simulink model "IEEE_BUS_68_AGC"  (R2025a)
settings: Solver=ode23tb  StartTime=0.0  StopTime=150  FixedStep=Ts  MaxStep=0.0001  RelTol=1e-3
PreLoadFcn:
  | PSSMODEL=1;
  | LPSS=0;
  | WAPSS=0;
  | WAPSS2=0;
  | Ts=50e-5;
InitFcn:
  | PSSMODEL=1;
  | LPSS=0;
  | WAPSS=0;
  | WAPSS2=0;
  | Ts=50e-5;
  | 
  | % Required data to 68 Bus benchmark
  | % clear
  | % clc
  | % Definition for the columns
  | % system base =100 MVA
  | 
  | %% Line data Format (line)
  | % All values are given on the same system base MVA
  | % 1: From bus
  | % 2: To bus
  | % 3: Resistance (pu)
  | % 4: Reactance  (pu)
  | % 5: Charge     (pu)
  | % 6: Transformer Tap Amplitute
  | % 7: base MVA
  | % 8: Nomonal Voltage (KV)
  | 
  | %1   2    3        4       5       6        7      8
  | line=[...
  | 1	54	0	     0.0181	  0	      1.025     100    13.8
  | 2	58	0	     0.025	  0	      1.070     100    13.8
  | 3	62	0	     0.02	  0	      1.070     100    13.8
  | 4	19	0.0007	 0.0142	  0	      1.070     100    13.8
  | 5	20	0.0009	 0.018	  0	      1.009     100    13.8
  | 6	22	0	     0.0143	  0	      1.025     100    13.8
  | 7	23	0.0005	 0.0272	  0	      0         100    13.8
  | 8	25	0.0006	 0.0232	  0	      1.025     100    13.8
  | 9	29	0.0008	 0.0156   0	      1.025     100    13.8
  | 10	31	0	     0.026	  0	      1.04      100    13.8
  | 11	32	0	     0.013	  0	      1.04      100    13.8
  | 12	36	0	     0.0075	  0	      1.04      100    13.8
  | 13	17	0	     0.0033	  0	      1.04      100    13.8
  | 14	41	0	     0.0015	  0	      1         100    13.8
  | 15	42	0	     0.0015	  0	      1         100    13.8
  | 16	18	0	     0.003	  0	      1         100    13.8
  | 17	36	0.0005	 0.0045	  0.32	  0         100    138
  | 17	43	0.0005	 0.0276	  0	      0         100    138
  | 18	42	0.004	 0.06	  2.25    0         100    138
  | 18	49	0.0076	 0.1141	  1.16    0	        100    138
  | 18	50	0.0012	 0.0288	  2.06	  0         100    138
  | 20	19	0.0007	 0.0138	  0       1.06	    100    138
  | 19	68	0.0016	 0.0195	  0.304	  0         100    138
  | 21	22	0.0008	 0.014	  0.2565  0	        100    138
  | 21	68	0.0008	 0.0135	  0.2548  0	        100    138
  | 22	23	0.0006	 0.0096	  0.1846  0	        100    138
  | 23	24	0.0022	 0.035	  0.361	  0         100    138
  | 24	68	0.0003	 0.0059	  0.068	  0         100    138
  | 25	26	0.0032	 0.0323	  0.531	  0         100    138
  | 25	54	0.007	 0.0086	  0.146	  0         100    138
  | 26	27	0.0014	 0.0147	  0.2396  0	        100    138
  | 26	28	0.0043	 0.0474	  0.7802  0	        100    138
  | 26	29	0.0057	 0.0625	  1.029	  0         100    138
  | 27	37	0.0013	 0.0173	  0.3216  0	        100    138
  | 27	53	0.032	 0.32	  0.41	  0         100    138
  | ... (+206 lines)
undefined symbols (not defined in the file or in its folder): D1, Delta
libraries: spsPMUPLLBasedPositiveSequenceLib x90, spsRMSLib x73, spsThreePhaseVIMeasurementLib x69, spsLoadFlowBusLib x69, spsThreePhasePISectionLineLib x64, spsThreePhaseParallelRLCLoadLib x35, spsGenericPowerSystemStabilizerLib x32, spsThreePhaseSeriesRLCLoadLib x21, spsThreePhaseTransformerTwoWindingsLib x21, spsSynchronousMachinepuStandardLib x20, spsExcitationSystemLib x16, spsMultiBandPowerSystemStabilizerLib x16
(part 8 of 8)

== system IEEE_BUS_68_AGC/area-4/G10/M10: Turbine & Regulators  ==
  note: M10
  m10 : Inport
  Pref10 : Inport  Port=2
  Vref10 : Inport  Port=3
  PSS10 : Inport  Port=4
  Bus Selector : BusSelector  OutputSignals="Mechanical.Rotor speed  wm  (pu),Mechanical.Rotor angle deviation  d_theta (rad),Mechanical.Electrical power  Pe (pu),Mechanical.Rotor speed deviation  dw (pu),Mechanical.Rotor mechanical angle  theta (deg),dq0 components.Stator voltage  vd (pu),dq0 components.Stator voltage  vq (pu),Output reactive power  Qeo (pu)"
  "Delta Pa PSS 10 " : spsGenericPowerSystemStabilizerLib/Generic Power System Stabilizer  Tsensor=15e-3  K=2.5*1.25  Twashout=1  Tleadlag1=[60e-3 1]  Tleadlag2=[0 0]  VSlimits=[-0.15 0.15]  Vinit=0  Plot_On=off  MagdB_On=on  FreqRange=logspace(-2,2,500)
      settings: LibrarySourceBlock=|
      | sps_lib/Electrical Machines/Synchronous Machine Control/Generic
      | Power System Stabilizer
  Delta w PSS (Kundur) 10 : spsGenericPowerSystemStabilizerLib/Generic Power System Stabilizer  Tsensor=15e-3  K=30  Twashout=10  Tleadlag1=[50e-3 20e-3]  Tleadlag2=[3 5.4]  VSlimits=[-0.15 0.15]  Vinit=0  Plot_On=off  MagdB_On=on  FreqRange=logspace(-2,2,500)
      settings: LibrarySourceBlock=|
      | sps_lib/Electrical Machines/Synchronous Machine Control/Generic
      | Power System Stabilizer
  EXCITATION10 : spsExcitationSystemLib/Excitation System  tr=AVR_Data(7,1)  reg=[ AVR_Data(7,2:3) ]  exc=[ 1, 0 ]  tgr=[ AVR_Data(7,4:5)]  damp=[ 0, 0 ]  sat=[ 0, 0 ]  lim="[ AVR_Data(7,7:8)  0 ]"  v0=[1.01 1.0142]
      settings: LibrarySourceBlock=sps_lib/Electrical Machines/Synchronous Machine Control/Excitation System
  MB-PSS10 : spsMultiBandPowerSystemStabilizerLib/Multi-Band Power System Stabilizer  OperationMode=Simplified settings  Kg=MB(1)  GL=[MB(2) MB(3)]  GI=[MB(4) MB(5)]  GH=[MB(6) MB(7)]  GLd=[66 66 9.4]  TcLF=[1.667 2 0 0 0 0 2 2.4 0 0 0 0 1 1]  GId=[66 66 47.6]  TcIF=[1 1 0.25 0.3 0 0 1 1 0.3 0.36 0 0 0 0]  GHd=[66 66 233]  TcHF="[0.01 0.012 0 0 0 0  0.012 0.0144 0 0 0 0 1 1]"  LIM=[.075 .15 .15 .15]  Plot_On=off  MagdB_On=off  FreqRange=logspace(-2,2,500)
      settings: LibrarySourceBlock=|
      | sps_lib/Electrical Machines/Synchronous Machine Control/Multi-Band
      | Power System Stabilizer
  Multiport Switch1 : MultiPortSwitch  Inputs=4  SaturateOnIntegerOverflow=off
  PSS model3 : Constant  Value=0
  PSS model4 : Constant
  Real-Imag to Complex1 : RealImagToComplex
  STG10 : spsSteamTurbineandGovernorLib/Steam Turbine and Governor  gentype=Tandem-compound (single mass)  reg1="[ 1  0.05    0 ]"  reg2="[ 0.001  0.15 ]"  reg3="[ -0.1  0.1  0  4.496 ]"  N=Ns  turb1="[ 0  10   3.3   0.5   ]"  turb2="[   0   0.36    0.36   0.28   ]"  HA="[ 0.046  1.430  1.465   0.192 ]"  KA="[ 90.44  53.88  64.59   62.94  ]"  DA="[ 0.0115  0.3575  0.3663   0.0137  ]"  ini1=0.5  ini2=[0.779316,-31.4247]
      settings: LibrarySourceBlock=|
      | sps_lib/Electrical Machines/Synchronous Machine Control/Steam Turbine
      | and Governor
  Sum2 : Sum  InputSameDT=on  SaturateOnIntegerOverflow=on  OutDataTypeStr=Inherit: Same as first input
  Sum3 : Sum  Inputs=-+  InputSameDT=on  SaturateOnIntegerOverflow=on  OutDataTypeStr=Inherit: Same as first input
  Terminator3 : Terminator
  Terminator4 : Terminator
  Terminator5 : Terminator
  wref10 : Constant
  Pm10 : Outport  InitialOutput=0
  Vf10 : Outport  Port=2  InitialOutput=0
  tag scope: EFD10=global, Pa10=global, Pe10=global, Q10=global, Vt10=global, d_theta10=global, pss10=global, theta10=global, w10=global
  wires:
  PSS10/1 -> Sum2/1
  Multiport Switch1/1 -> EXCITATION10/4, [pss10]
  PSS model3/1 -> Multiport Switch1/2
  MB-PSS10/1 -> Multiport Switch1/3
  Delta w PSS (Kundur) 10/1 -> Multiport Switch1/4
  "Delta Pa PSS 10 "/1 -> Multiport Switch1/5
  PSS model4/1 -> Sum2/2
  Sum2/1 -> Multiport Switch1/1
  Sum3/1 -> "Delta Pa PSS 10 "/1, [Pa10]  "Pm-Pe"
  Bus Selector/8 -> [Q10]  "<Output reactive power  Qeo (pu)>"
  Bus Selector/4 -> MB-PSS10/1, Delta w PSS (Kundur) 10/1  "<Rotor speed deviation  dw (pu)>"
  Bus Selector/3 -> [Pe10], Sum3/1  "<Electrical power  Pe (pu)>"
  Bus Selector/2 -> [d_theta10], STG10/4  "<Rotor angle deviation  d_theta (rad)>"
  Bus Selector/1 -> STG10/3, [w10]  "<Rotor speed  wm  (pu)>"
  STG10/1 -> Terminator5/1
  STG10/2 -> Terminator4/1
  STG10/4 -> Pm10/1, Sum3/2
  STG10/3 -> Terminator3/1
  Bus Selector/6 -> Real-Imag to Complex1/1, EXCITATION10/2  "<Stator voltage  vd (pu)>"
  Bus Selector/5 -> [theta10]  "<Rotor mechanical angle  theta (deg)>"
  Real-Imag to Complex1/1 -> [Vt10]
  EXCITATION10/1 -> [EFD10], Vf10/1
  Vref10/1 -> EXCITATION10/1
  m10/1 -> Bus Selector/1
  Pref10/1 -> STG10/2
  wref10/1 -> STG10/1
  Bus Selector/7 -> Real-Imag to Complex1/2, EXCITATION10/3  "<Stator voltage  vq (pu)>"

== system IEEE_BUS_68_AGC/area-4/G11/M11: Turbine & Regulators  ==
  note: M11
  m11 : Inport
  Pref11 : Inport  Port=2
  Vref11 : Inport  Port=3
  PSS11 : Inport  Port=4
  Bus Selector : BusSelector  OutputSignals="Mechanical.Rotor speed  wm  (pu),Mechanical.Rotor angle deviation  d_theta (rad),Mechanical.Electrical power  Pe (pu),Mechanical.Rotor speed deviation  dw (pu),Mechanical.Rotor mechanical angle  theta (deg),dq0 components.Stator voltage  vd (pu),dq0 components.Stator voltage  vq (pu),Output reactive power  Qeo (pu)"
  "Delta Pa PSS 11 " : spsGenericPowerSystemStabilizerLib/Generic Power System Stabilizer  Tsensor=15e-3  K=2.5*1.25  Twashout=1  Tleadlag1=[60e-3 1]  Tleadlag2=[0 0]  VSlimits=[-0.15 0.15]  Vinit=0  Plot_On=off  MagdB_On=on  FreqRange=logspace(-2,2,500)
      settings: LibrarySourceBlock=|
      | sps_lib/Electrical Machines/Synchronous Machine Control/Generic
      | Power System Stabilizer
  Delta w PSS (Kundur) 11 : spsGenericPowerSystemStabilizerLib/Generic Power System Stabilizer  Tsensor=15e-3  K=30  Twashout=10  Tleadlag1=[50e-3 20e-3]  Tleadlag2=[3 5.4]  VSlimits=[-0.15 0.15]  Vinit=0  Plot_On=off  MagdB_On=on  FreqRange=logspace(-2,2,500)
      settings: LibrarySourceBlock=|
      | sps_lib/Electrical Machines/Synchronous Machine Control/Generic
      | Power System Stabilizer
  EXCITATION11 : spsExcitationSystemLib/Excitation System  tr=AVR_Data(11,1)  reg=[ AVR_Data(11,2:3) ]  exc=[ 1, 0 ]  tgr=[ AVR_Data(11,4:5)]  damp=[ 0, 0 ]  sat=[ 0, 0 ]  lim="[ AVR_Data(11,7:8)  0 ]"  v0=[1 1.0051]
      settings: LibrarySourceBlock=sps_lib/Electrical Machines/Synchronous Machine Control/Excitation System
  MB-PSS11 : spsMultiBandPowerSystemStabilizerLib/Multi-Band Power System Stabilizer  OperationMode=Simplified settings  Kg=MB(1)  GL=[MB(2) MB(3)]  GI=[MB(4) MB(5)]  GH=[MB(6) MB(7)]  GLd=[66 66 9.4]  TcLF=[1.667 2 0 0 0 0 2 2.4 0 0 0 0 1 1]  GId=[66 66 47.6]  TcIF=[1 1 0.25 0.3 0 0 1 1 0.3 0.36 0 0 0 0]  GHd=[66 66 233]  TcHF="[0.01 0.012 0 0 0 0  0.012 0.0144 0 0 0 0 1 1]"  LIM=[.075 .15 .15 .15]  Plot_On=off  MagdB_On=off  FreqRange=logspace(-2,2,500)
      settings: LibrarySourceBlock=|
      | sps_lib/Electrical Machines/Synchronous Machine Control/Multi-Band
      | Power System Stabilizer
  Multiport Switch1 : MultiPortSwitch  Inputs=4  SaturateOnIntegerOverflow=off
  PSS model3 : Constant  Value=0
  PSS model4 : Constant
  Real-Imag to Complex1 : RealImagToComplex
  STG11 : spsSteamTurbineandGovernorLib/Steam Turbine and Governor  gentype=Tandem-compound (single mass)  reg1="[ 1  0.05    0 ]"  reg2="[ 0.001  0.15 ]"  reg3="[ -0.1  0.1  0  4.496 ]"  N=Ns  turb1="[ 0  10   3.3   0.5   ]"  turb2="[   0   0.36    0.36   0.28   ]"  HA="[ 0.046  1.430  1.465   0.192 ]"  KA="[ 90.44  53.88  64.59   62.94  ]"  DA="[ 0.0115  0.3575  0.3663   0.0137  ]"  ini1=0.5  ini2=[0.779316,-31.4247]
      settings: LibrarySourceBlock=|
      | sps_lib/Electrical Machines/Synchronous Machine Control/Steam Turbine
      | and Governor
  Sum2 : Sum  InputSameDT=on  SaturateOnIntegerOverflow=on  OutDataTypeStr=Inherit: Same as first input
  Sum3 : Sum  Inputs=-+  InputSameDT=on  SaturateOnIntegerOverflow=on  OutDataTypeStr=Inherit: Same as first input
  Terminator3 : Terminator
  Terminator4 : Terminator
  Terminator5 : Terminator
  wref11 : Constant
  Pm11 : Outport  InitialOutput=0
  Vf11 : Outport  Port=2  InitialOutput=0
  tag scope: EFD11=global, Pa11=global, Pe11=global, Q11=global, Vt11=global, d_theta11=global, pss11=global, theta11=global, w11=global
  wires:
  Bus Selector/7 -> EXCITATION11/3, Real-Imag to Complex1/2  "<Stator voltage  vq (pu)>"
  wref11/1 -> STG11/1
  Pref11/1 -> STG11/2
  m11/1 -> Bus Selector/1
  Vref11/1 -> EXCITATION11/1
  EXCITATION11/1 -> Vf11/1, [EFD11]
  Real-Imag to Complex1/1 -> [Vt11]
  Bus Selector/5 -> [theta11]  "<Rotor mechanical angle  theta (deg)>"
  Bus Selector/6 -> EXCITATION11/2, Real-Imag to Complex1/1  "<Stator voltage  vd (pu)>"
  STG11/3 -> Terminator3/1
  STG11/4 -> Sum3/2, Pm11/1
  STG11/2 -> Terminator4/1
  STG11/1 -> Terminator5/1
  Bus Selector/1 -> [w11], STG11/3  "<Rotor speed  wm  (pu)>"
  Bus Selector/2 -> STG11/4, [d_theta11]  "<Rotor angle deviation  d_theta (rad)>"
  Bus Selector/3 -> Sum3/1, [Pe11]  "<Electrical power  Pe (pu)>"
  Bus Selector/4 -> Delta w PSS (Kundur) 11/1, MB-PSS11/1  "<Rotor speed deviation  dw (pu)>"
  Bus Selector/8 -> [Q11]  "<Output reactive power  Qeo (pu)>"
  Sum3/1 -> [Pa11], "Delta Pa PSS 11 "/1  "Pm-Pe"
  Sum2/1 -> Multiport Switch1/1
  PSS model4/1 -> Sum2/2
  "Delta Pa PSS 11 "/1 -> Multiport Switch1/5
  Delta w PSS (Kundur) 11/1 -> Multiport Switch1/4
  MB-PSS11/1 -> Multiport Switch1/3
  PSS model3/1 -> Multiport Switch1/2
  Multiport Switch1/1 -> [pss11], EXCITATION11/4
  PSS11/1 -> Sum2/1

== system IEEE_BUS_68_AGC/area-4/G12/M12: Turbine & Regulators  ==
  note: M12
  m12 : Inport
  Pref12 : Inport  Port=2
  Vref12 : Inport  Port=3
  PSS12 : Inport  Port=4
  Bus Selector : BusSelector  OutputSignals="Mechanical.Rotor speed  wm  (pu),Mechanical.Rotor angle deviation  d_theta (rad),Mechanical.Electrical power  Pe (pu),Mechanical.Rotor speed deviation  dw (pu),Mechanical.Rotor mechanical angle  theta (deg),dq0 components.Stator voltage  vd (pu),dq0 components.Stator voltage  vq (pu),Output reactive power  Qeo (pu)"
  "Delta Pa PSS 12 " : spsGenericPowerSystemStabilizerLib/Generic Power System Stabilizer  Tsensor=15e-3  K=2.5*1.25  Twashout=1  Tleadlag1=[60e-3 1]  Tleadlag2=[0 0]  VSlimits=[-0.15 0.15]  Vinit=0  Plot_On=off  MagdB_On=on  FreqRange=logspace(-2,2,500)
      settings: LibrarySourceBlock=|
      | sps_lib/Electrical Machines/Synchronous Machine Control/Generic
      | Power System Stabilizer
  Delta w PSS (Kundur) 12 : spsGenericPowerSystemStabilizerLib/Generic Power System Stabilizer  Tsensor=15e-3  K=30  Twashout=10  Tleadlag1=[50e-3 20e-3]  Tleadlag2=[3 5.4]  VSlimits=[-0.15 0.15]  Vinit=0  Plot_On=off  MagdB_On=on  FreqRange=logspace(-2,2,500)
      settings: LibrarySourceBlock=|
      | sps_lib/Electrical Machines/Synchronous Machine Control/Generic
      | Power System Stabilizer
  EXCITATION12 : spsExcitationSystemLib/Excitation System  tr=AVR_Data(13,1)  reg=[ AVR_Data(13,2:3) ]  exc=[ 1, 0 ]  tgr=[ AVR_Data(13,4:5)]  damp=[ 0, 0 ]  sat=[ 0, 0 ]  lim="[ AVR_Data(13,7:8)  0 ]"  v0=[1.0156 1.0136]
      settings: LibrarySourceBlock=sps_lib/Electrical Machines/Synchronous Machine Control/Excitation System
  MB-PSS12 : spsMultiBandPowerSystemStabilizerLib/Multi-Band Power System Stabilizer  OperationMode=Simplified settings  Kg=MB(1)  GL=[MB(2) MB(3)]  GI=[MB(4) MB(5)]  GH=[MB(6) MB(7)]  GLd=[66 66 9.4]  TcLF=[1.667 2 0 0 0 0 2 2.4 0 0 0 0 1 1]  GId=[66 66 47.6]  TcIF=[1 1 0.25 0.3 0 0 1 1 0.3 0.36 0 0 0 0]  GHd=[66 66 233]  TcHF="[0.01 0.012 0 0 0 0  0.012 0.0144 0 0 0 0 1 1]"  LIM=[.075 .15 .15 .15]  Plot_On=off  MagdB_On=off  FreqRange=logspace(-2,2,500)
      settings: LibrarySourceBlock=|
      | sps_lib/Electrical Machines/Synchronous Machine Control/Multi-Band
      | Power System Stabilizer
  Multiport Switch1 : MultiPortSwitch  Inputs=4  SaturateOnIntegerOverflow=off
  PSS model3 : Constant  Value=0
  PSS model4 : Constant
  Real-Imag to Complex1 : RealImagToComplex
  STG12 : spsSteamTurbineandGovernorLib/Steam Turbine and Governor  gentype=Tandem-compound (single mass)  reg1="[ 1  0.05    0 ]"  reg2="[ 0.001  0.15 ]"  reg3="[ -0.1  0.1  0  4.496 ]"  N=Ns  turb1="[ 0  10   3.3   0.5   ]"  turb2="[   0   0.36    0.36   0.28   ]"  HA="[ 0.046  1.430  1.465   0.192 ]"  KA="[ 90.44  53.88  64.59   62.94  ]"  DA="[ 0.0115  0.3575  0.3663   0.0137  ]"  ini1=0.45  ini2=[0.779316,-31.4247]
      settings: LibrarySourceBlock=|
      | sps_lib/Electrical Machines/Synchronous Machine Control/Steam Turbine
      | and Governor
  Sum2 : Sum  InputSameDT=on  SaturateOnIntegerOverflow=on  OutDataTypeStr=Inherit: Same as first input
  Sum3 : Sum  Inputs=-+  InputSameDT=on  SaturateOnIntegerOverflow=on  OutDataTypeStr=Inherit: Same as first input
  Terminator3 : Terminator
  Terminator4 : Terminator
  Terminator5 : Terminator
  wref12 : Constant
  Pm12 : Outport  InitialOutput=0
  Vf12 : Outport  Port=2  InitialOutput=0
  tag scope: EFD12=global, Pa12=global, Pe12=global, Q12=global, Vt12=global, d_theta12=global, pss12=global, theta12=global, w12=global
  wires:
  PSS12/1 -> Sum2/1
  Multiport Switch1/1 -> EXCITATION12/4, [pss12]
  PSS model3/1 -> Multiport Switch1/2
  MB-PSS12/1 -> Multiport Switch1/3
  Delta w PSS (Kundur) 12/1 -> Multiport Switch1/4
  "Delta Pa PSS 12 "/1 -> Multiport Switch1/5
  PSS model4/1 -> Sum2/2
  Sum2/1 -> Multiport Switch1/1
  Sum3/1 -> "Delta Pa PSS 12 "/1, [Pa12]  "Pm-Pe"
  Bus Selector/8 -> [Q12]  "<Output reactive power  Qeo (pu)>"
  Bus Selector/4 -> MB-PSS12/1, Delta w PSS (Kundur) 12/1  "<Rotor speed deviation  dw (pu)>"
  Bus Selector/3 -> [Pe12], Sum3/1  "<Electrical power  Pe (pu)>"
  Bus Selector/2 -> [d_theta12], STG12/4  "<Rotor angle deviation  d_theta (rad)>"
  Bus Selector/1 -> STG12/3, [w12]  "<Rotor speed  wm  (pu)>"
  STG12/1 -> Terminator5/1
  STG12/2 -> Terminator4/1
  STG12/4 -> Pm12/1, Sum3/2
  STG12/3 -> Terminator3/1
  Bus Selector/6 -> Real-Imag to Complex1/1, EXCITATION12/2  "<Stator voltage  vd (pu)>"
  Bus Selector/5 -> [theta12]  "<Rotor mechanical angle  theta (deg)>"
  Real-Imag to Complex1/1 -> [Vt12]
  EXCITATION12/1 -> [EFD12], Vf12/1
  Vref12/1 -> EXCITATION12/1
  m12/1 -> Bus Selector/1
  Pref12/1 -> STG12/2
  wref12/1 -> STG12/1
  Bus Selector/7 -> Real-Imag to Complex1/2, EXCITATION12/3  "<Stator voltage  vq (pu)>"

== system IEEE_BUS_68_AGC/area-4/G13/M13: Turbine & Regulators  ==
  note: M13
  m13 : Inport
  Pref13 : Inport  Port=2
  Vref13 : Inport  Port=3
  PSS13 : Inport  Port=4
  Bus Selector : BusSelector  OutputSignals="Mechanical.Rotor speed  wm  (pu),Mechanical.Rotor angle deviation  d_theta (rad),Mechanical.Electrical power  Pe (pu),Mechanical.Rotor speed deviation  dw (pu),Mechanical.Rotor mechanical angle  theta (deg),dq0 components.Stator voltage  vd (pu),dq0 components.Stator voltage  vq (pu),Output reactive power  Qeo (pu)"
  "Delta Pa PSS 13 " : spsGenericPowerSystemStabilizerLib/Generic Power System Stabilizer  Tsensor=15e-3  K=2.5*1.25  Twashout=1  Tleadlag1=[60e-3 1]  Tleadlag2=[0 0]  VSlimits=[-0.15 0.15]  Vinit=0  Plot_On=off  MagdB_On=on  FreqRange=logspace(-2,2,500)
      settings: LibrarySourceBlock=|
      | sps_lib/Electrical Machines/Synchronous Machine Control/Generic
      | Power System Stabilizer
  Delta w PSS (Kundur) 13 : spsGenericPowerSystemStabilizerLib/Generic Power System Stabilizer  Tsensor=15e-3  K=30  Twashout=10  Tleadlag1=[50e-3 20e-3]  Tleadlag2=[3 5.4]  VSlimits=[-0.15 0.15]  Vinit=0  Plot_On=off  MagdB_On=on  FreqRange=logspace(-2,2,500)
      settings: LibrarySourceBlock=|
      | sps_lib/Electrical Machines/Synchronous Machine Control/Generic
      | Power System Stabilizer
  EXCITATION13 : spsExcitationSystemLib/Excitation System  tr=AVR_Data(13,1)  reg=[ AVR_Data(13,2:3) ]  exc=[ 1, 0 ]  tgr=[ AVR_Data(13,4:5)]  damp=[ 0, 0 ]  sat=[ 0, 0 ]  lim="[ AVR_Data(13,7:8)  0 ]"  v0=[1.011 1.016]
      settings: LibrarySourceBlock=sps_lib/Electrical Machines/Synchronous Machine Control/Excitation System
  MB-PSS13 : spsMultiBandPowerSystemStabilizerLib/Multi-Band Power System Stabilizer  OperationMode=Simplified settings  Kg=MB(1)  GL=[MB(2) MB(3)]  GI=[MB(4) MB(5)]  GH=[MB(6) MB(7)]  GLd=[66 66 9.4]  TcLF=[1.667 2 0 0 0 0 2 2.4 0 0 0 0 1 1]  GId=[66 66 47.6]  TcIF=[1 1 0.25 0.3 0 0 1 1 0.3 0.36 0 0 0 0]  GHd=[66 66 233]  TcHF="[0.01 0.012 0 0 0 0  0.012 0.0144 0 0 0 0 1 1]"  LIM=[.075 .15 .15 .15]  Plot_On=off  MagdB_On=off  FreqRange=logspace(-2,2,500)
      settings: LibrarySourceBlock=|
      | sps_lib/Electrical Machines/Synchronous Machine Control/Multi-Band
      | Power System Stabilizer
  Multiport Switch1 : MultiPortSwitch  Inputs=4  SaturateOnIntegerOverflow=off
  PSS model3 : Constant  Value=0
  PSS model4 : Constant
  Real-Imag to Complex1 : RealImagToComplex
  STG13 : spsSteamTurbineandGovernorLib/Steam Turbine and Governor  gentype=Tandem-compound (single mass)  reg1="[ 1  0.05    0 ]"  reg2="[ 0.001  0.15 ]"  reg3="[ -0.1  0.1  0  4.496 ]"  N=Ns  turb1="[ 0  10   3.3   0.5   ]"  turb2="[   0   0.36    0.36   0.28   ]"  HA="[ 0.046  1.430  1.465   0.192 ]"  KA="[ 90.44  53.88  64.59   62.94  ]"  DA="[ 0.0115  0.3575  0.3663   0.0137  ]"  ini1=0.5985  ini2=[0.779316,-31.4247]
      settings: LibrarySourceBlock=|
      | sps_lib/Electrical Machines/Synchronous Machine Control/Steam Turbine
      | and Governor
  Sum2 : Sum  InputSameDT=on  SaturateOnIntegerOverflow=on  OutDataTypeStr=Inherit: Same as first input
  Sum3 : Sum  Inputs=-+  InputSameDT=on  SaturateOnIntegerOverflow=on  OutDataTypeStr=Inherit: Same as first input
  Terminator3 : Terminator
  Terminator4 : Terminator
  Terminator5 : Terminator
  wref13 : Constant
  Pm13 : Outport  InitialOutput=0
  Vf13 : Outport  Port=2  InitialOutput=0
  tag scope: EFD13=global, Pa13=global, Pe13=global, Q13=global, Vt13=global, d_theta13=global, pss13=global, theta13=global, w13=global
  wires:
  Bus Selector/7 -> EXCITATION13/3, Real-Imag to Complex1/2  "<Stator voltage  vq (pu)>"
  wref13/1 -> STG13/1
  Pref13/1 -> STG13/2
  m13/1 -> Bus Selector/1
  Vref13/1 -> EXCITATION13/1
  EXCITATION13/1 -> Vf13/1, [EFD13]
  Real-Imag to Complex1/1 -> [Vt13]
  Bus Selector/5 -> [theta13]  "<Rotor mechanical angle  theta (deg)>"
  Bus Selector/6 -> EXCITATION13/2, Real-Imag to Complex1/1  "<Stator voltage  vd (pu)>"
  STG13/3 -> Terminator3/1
  STG13/4 -> Sum3/2, Pm13/1
  STG13/2 -> Terminator4/1
  STG13/1 -> Terminator5/1
  Bus Selector/1 -> [w13], STG13/3  "<Rotor speed  wm  (pu)>"
  Bus Selector/2 -> STG13/4, [d_theta13]  "<Rotor angle deviation  d_theta (rad)>"
  Bus Selector/3 -> Sum3/1, [Pe13]  "<Electrical power  Pe (pu)>"
  Bus Selector/4 -> Delta w PSS (Kundur) 13/1, MB-PSS13/1  "<Rotor speed deviation  dw (pu)>"
  Bus Selector/8 -> [Q13]  "<Output reactive power  Qeo (pu)>"
  Sum3/1 -> [Pa13], "Delta Pa PSS 13 "/1  "Pm-Pe"
  Sum2/1 -> Multiport Switch1/1
  PSS model4/1 -> Sum2/2
  "Delta Pa PSS 13 "/1 -> Multiport Switch1/5
  Delta w PSS (Kundur) 13/1 -> Multiport Switch1/4
  MB-PSS13/1 -> Multiport Switch1/3
  PSS model3/1 -> Multiport Switch1/2
  Multiport Switch1/1 -> [pss13], EXCITATION13/4
  PSS13/1 -> Sum2/1

== system IEEE_BUS_68_AGC/area-5/G14/M14: Turbine & Regulators  ==
  note: M14
  m14 : Inport
  Pref14 : Inport  Port=2
  Vref14 : Inport  Port=3
  PSS14 : Inport  Port=4
  Bus Selector : BusSelector  OutputSignals="Mechanical.Rotor speed  wm  (pu),Mechanical.Rotor angle deviation  d_theta (rad),Mechanical.Electrical power  Pe (pu),Mechanical.Rotor speed deviation  dw (pu),Mechanical.Rotor mechanical angle  theta (deg),dq0 components.Stator voltage  vd (pu),dq0 components.Stator voltage  vq (pu),Output reactive power  Qeo (pu)"
  "Delta Pa PSS 14 " : spsGenericPowerSystemStabilizerLib/Generic Power System Stabilizer  Tsensor=15e-3  K=2.5*1.25  Twashout=1  Tleadlag1=[60e-3 1]  Tleadlag2=[0 0]  VSlimits=[-0.15 0.15]  Vinit=0  Plot_On=off  MagdB_On=on  FreqRange=logspace(-2,2,500)
      settings: LibrarySourceBlock=|
      | sps_lib/Electrical Machines/Synchronous Machine Control/Generic
      | Power System Stabilizer
  Delta w PSS (Kundur) 14 : spsGenericPowerSystemStabilizerLib/Generic Power System Stabilizer  Tsensor=15e-3  K=30  Twashout=10  Tleadlag1=[50e-3 20e-3]  Tleadlag2=[3 5.4]  VSlimits=[-0.15 0.15]  Vinit=0  Plot_On=off  MagdB_On=on  FreqRange=logspace(-2,2,500)
      settings: LibrarySourceBlock=|
      | sps_lib/Electrical Machines/Synchronous Machine Control/Generic
      | Power System Stabilizer
  EXCITATION14 : spsExcitationSystemLib/Excitation System  tr=AVR_Data(14,1)  reg=[ AVR_Data(14,2:3) ]  exc=[ 1, 0 ]  tgr=[ AVR_Data(14,4:5)]  damp=[ 0, 0 ]  sat=[ 0, 0 ]  lim="[ AVR_Data(14,7:8)  0 ]"  v0=[1 1.0004]
      settings: LibrarySourceBlock=sps_lib/Electrical Machines/Synchronous Machine Control/Excitation System
  MB-PSS14 : spsMultiBandPowerSystemStabilizerLib/Multi-Band Power System Stabilizer  OperationMode=Simplified settings  Kg=MB(1)  GL=[MB(2) MB(3)]  GI=[MB(4) MB(5)]  GH=[MB(6) MB(7)]  GLd=[66 66 9.4]  TcLF=[1.667 2 0 0 0 0 2 2.4 0 0 0 0 1 1]  GId=[66 66 47.6]  TcIF=[1 1 0.25 0.3 0 0 1 1 0.3 0.36 0 0 0 0]  GHd=[66 66 233]  TcHF="[0.01 0.012 0 0 0 0  0.012 0.0144 0 0 0 0 1 1]"  LIM=[.075 .15 .15 .15]  Plot_On=off  MagdB_On=off  FreqRange=logspace(-2,2,500)
      settings: LibrarySourceBlock=|
      | sps_lib/Electrical Machines/Synchronous Machine Control/Multi-Band
      | Power System Stabilizer
  Multiport Switch1 : MultiPortSwitch  Inputs=4  SaturateOnIntegerOverflow=off
  PSS model3 : Constant  Value=0
  PSS model4 : Constant
  Real-Imag to Complex1 : RealImagToComplex
  STG14 : spsSteamTurbineandGovernorLib/Steam Turbine and Governor  gentype=Tandem-compound (single mass)  reg1="[ 1  0.05    0 ]"  reg2="[ 0.001  0.15 ]"  reg3="[ -0.1  0.1  0  4.496 ]"  N=Ns  turb1="[ 0  10   3.3   0.5   ]"  turb2="[   0   0.36    0.36   0.28   ]"  HA="[ 0.046  1.430  1.465   0.192 ]"  KA="[ 90.44  53.88  64.59   62.94  ]"  DA="[ 0.0115  0.3575  0.3663   0.0137  ]"  ini1=0.595  ini2=[0.779316,-31.4247]
      settings: LibrarySourceBlock=|
      | sps_lib/Electrical Machines/Synchronous Machine Control/Steam Turbine
      | and Governor
  Sum2 : Sum  InputSameDT=on  SaturateOnIntegerOverflow=on  OutDataTypeStr=Inherit: Same as first input
  Sum3 : Sum  Inputs=-+  InputSameDT=on  SaturateOnIntegerOverflow=on  OutDataTypeStr=Inherit: Same as first input
  Terminator3 : Terminator
  Terminator4 : Terminator
  Terminator5 : Terminator
  wref14 : Constant
  Pm14 : Outport  InitialOutput=0
  Vf14 : Outport  Port=2  InitialOutput=0
  tag scope: EFD14=global, Pa14=global, Pe14=global, Q14=global, Vt14=global, d_theta14=global, pss14=global, theta14=global, w14=global
  wires:
  PSS14/1 -> Sum2/1
  Multiport Switch1/1 -> EXCITATION14/4, [pss14]
  PSS model3/1 -> Multiport Switch1/2
  MB-PSS14/1 -> Multiport Switch1/3
  Delta w PSS (Kundur) 14/1 -> Multiport Switch1/4
  "Delta Pa PSS 14 "/1 -> Multiport Switch1/5
  PSS model4/1 -> Sum2/2
  Sum2/1 -> Multiport Switch1/1
  Sum3/1 -> "Delta Pa PSS 14 "/1, [Pa14]  "Pm-Pe"
  Bus Selector/8 -> [Q14]  "<Output reactive power  Qeo (pu)>"
  Bus Selector/4 -> MB-PSS14/1, Delta w PSS (Kundur) 14/1  "<Rotor speed deviation  dw (pu)>"
  Bus Selector/3 -> [Pe14], Sum3/1  "<Electrical power  Pe (pu)>"
  Bus Selector/2 -> [d_theta14], STG14/4  "<Rotor angle deviation  d_theta (rad)>"
  Bus Selector/1 -> STG14/3, [w14]  "<Rotor speed  wm  (pu)>"
  STG14/1 -> Terminator5/1
  STG14/2 -> Terminator4/1
  STG14/4 -> Pm14/1, Sum3/2
  STG14/3 -> Terminator3/1
  Bus Selector/6 -> Real-Imag to Complex1/1, EXCITATION14/2  "<Stator voltage  vd (pu)>"
  Bus Selector/5 -> [theta14]  "<Rotor mechanical angle  theta (deg)>"
  Real-Imag to Complex1/1 -> [Vt14]
  EXCITATION14/1 -> [EFD14], Vf14/1
  Vref14/1 -> EXCITATION14/1
  m14/1 -> Bus Selector/1
  Pref14/1 -> STG14/2
  wref14/1 -> STG14/1
  Bus Selector/7 -> Real-Imag to Complex1/2, EXCITATION14/3  "<Stator voltage  vq (pu)>"

== system IEEE_BUS_68_AGC/area-5/G15/M15: Turbine & Regulators  ==
  note: M15
  m15 : Inport
  Pref15 : Inport  Port=2
  Vref15 : Inport  Port=3
  PSS15 : Inport  Port=4
  Bus Selector : BusSelector  OutputSignals="Mechanical.Rotor speed  wm  (pu),Mechanical.Rotor angle deviation  d_theta (rad),Mechanical.Electrical power  Pe (pu),Mechanical.Rotor speed deviation  dw (pu),Mechanical.Rotor mechanical angle  theta (deg),dq0 components.Stator voltage  vd (pu),dq0 components.Stator voltage  vq (pu),Output reactive power  Qeo (pu)"
  "Delta Pa PSS 15 " : spsGenericPowerSystemStabilizerLib/Generic Power System Stabilizer  Tsensor=15e-3  K=2.5*1.25  Twashout=1  Tleadlag1=[60e-3 1]  Tleadlag2=[0 0]  VSlimits=[-0.15 0.15]  Vinit=0  Plot_On=off  MagdB_On=on  FreqRange=logspace(-2,2,500)
      settings: LibrarySourceBlock=|
      | sps_lib/Electrical Machines/Synchronous Machine Control/Generic
      | Power System Stabilizer
  Delta w PSS (Kundur) 15 : spsGenericPowerSystemStabilizerLib/Generic Power System Stabilizer  Tsensor=15e-3  K=30  Twashout=10  Tleadlag1=[50e-3 20e-3]  Tleadlag2=[3 5.4]  VSlimits=[-0.15 0.15]  Vinit=0  Plot_On=off  MagdB_On=on  FreqRange=logspace(-2,2,500)
      settings: LibrarySourceBlock=|
      | sps_lib/Electrical Machines/Synchronous Machine Control/Generic
      | Power System Stabilizer
  EXCITATION15 : spsExcitationSystemLib/Excitation System  tr=AVR_Data(16,1)  reg=[ AVR_Data(16,2:3) ]  exc=[ 1, 0 ]  tgr=[ AVR_Data(16,4:5)]  damp=[ 0, 0 ]  sat=[ 0, 0 ]  lim="[ AVR_Data(16,7:8)  0 ]"  v0=[1 1.0003]
      settings: LibrarySourceBlock=sps_lib/Electrical Machines/Synchronous Machine Control/Excitation System
  MB-PSS15 : spsMultiBandPowerSystemStabilizerLib/Multi-Band Power System Stabilizer  OperationMode=Simplified settings  Kg=MB(1)  GL=[MB(2) MB(3)]  GI=[MB(4) MB(5)]  GH=[MB(6) MB(7)]  GLd=[66 66 9.4]  TcLF=[1.667 2 0 0 0 0 2 2.4 0 0 0 0 1 1]  GId=[66 66 47.6]  TcIF=[1 1 0.25 0.3 0 0 1 1 0.3 0.36 0 0 0 0]  GHd=[66 66 233]  TcHF="[0.01 0.012 0 0 0 0  0.012 0.0144 0 0 0 0 1 1]"  LIM=[.075 .15 .15 .15]  Plot_On=off  MagdB_On=off  FreqRange=logspace(-2,2,500)
      settings: LibrarySourceBlock=|
      | sps_lib/Electrical Machines/Synchronous Machine Control/Multi-Band
      | Power System Stabilizer
  Multiport Switch1 : MultiPortSwitch  Inputs=4  SaturateOnIntegerOverflow=off
  PSS model3 : Constant  Value=0
  PSS model4 : Constant
  Real-Imag to Complex1 : RealImagToComplex
  STG15 : spsSteamTurbineandGovernorLib/Steam Turbine and Governor  gentype=Tandem-compound (single mass)  reg1="[ 1  0.05    0 ]"  reg2="[ 0.001  0.15 ]"  reg3="[ -0.1  0.1  0  4.496 ]"  N=Ns  turb1="[ 0  10   3.3   0.5   ]"  turb2="[   0   0.36    0.36   0.28   ]"  HA="[ 0.046  1.430  1.465   0.192 ]"  KA="[ 90.44  53.88  64.59   62.94  ]"  DA="[ 0.0115  0.3575  0.3663   0.0137  ]"  ini1=0.33333  ini2=[0.779316,-31.4247]
      settings: LibrarySourceBlock=|
      | sps_lib/Electrical Machines/Synchronous Machine Control/Steam Turbine
      | and Governor
  Sum2 : Sum  InputSameDT=on  SaturateOnIntegerOverflow=on  OutDataTypeStr=Inherit: Same as first input
  Sum3 : Sum  Inputs=-+  InputSameDT=on  SaturateOnIntegerOverflow=on  OutDataTypeStr=Inherit: Same as first input
  Terminator3 : Terminator
  Terminator4 : Terminator
  Terminator5 : Terminator
  wref15 : Constant
  Pm15 : Outport  InitialOutput=0
  Vf15 : Outport  Port=2  InitialOutput=0
  tag scope: EFD15=global, Pa15=global, Pe15=global, Q15=global, Vt15=global, d_theta15=global, pss15=global, theta15=global, w15=global
  wires:
  Bus Selector/7 -> EXCITATION15/3, Real-Imag to Complex1/2  "<Stator voltage  vq (pu)>"
  wref15/1 -> STG15/1
  Pref15/1 -> STG15/2
  m15/1 -> Bus Selector/1
  Vref15/1 -> EXCITATION15/1
  EXCITATION15/1 -> Vf15/1, [EFD15]
  Real-Imag to Complex1/1 -> [Vt15]
  Bus Selector/5 -> [theta15]  "<Rotor mechanical angle  theta (deg)>"
  Bus Selector/6 -> EXCITATION15/2, Real-Imag to Complex1/1  "<Stator voltage  vd (pu)>"
  STG15/3 -> Terminator3/1
  STG15/4 -> Sum3/2, Pm15/1
  STG15/2 -> Terminator4/1
  STG15/1 -> Terminator5/1
  Bus Selector/1 -> [w15], STG15/3  "<Rotor speed  wm  (pu)>"
  Bus Selector/2 -> STG15/4, [d_theta15]  "<Rotor angle deviation  d_theta (rad)>"
  Bus Selector/3 -> Sum3/1, [Pe15]  "<Electrical power  Pe (pu)>"
  Bus Selector/4 -> Delta w PSS (Kundur) 15/1, MB-PSS15/1  "<Rotor speed deviation  dw (pu)>"
  Bus Selector/8 -> [Q15]  "<Output reactive power  Qeo (pu)>"
  Sum3/1 -> [Pa15], "Delta Pa PSS 15 "/1  "Pm-Pe"
  Sum2/1 -> Multiport Switch1/1
  PSS model4/1 -> Sum2/2
  "Delta Pa PSS 15 "/1 -> Multiport Switch1/5
  Delta w PSS (Kundur) 15/1 -> Multiport Switch1/4
  MB-PSS15/1 -> Multiport Switch1/3
  PSS model3/1 -> Multiport Switch1/2
  Multiport Switch1/1 -> [pss15], EXCITATION15/4
  PSS15/1 -> Sum2/1

== system IEEE_BUS_68_AGC/area-5/G16/M16: Turbine & Regulators  ==
  note: M16
  m16 : Inport
  Pref16 : Inport  Port=2
  Vref16 : Inport  Port=3
  PSS16 : Inport  Port=4
  Bus Selector : BusSelector  OutputSignals="Mechanical.Rotor speed  wm  (pu),Mechanical.Rotor angle deviation  d_theta (rad),Mechanical.Electrical power  Pe (pu),Mechanical.Rotor speed deviation  dw (pu),Mechanical.Rotor mechanical angle  theta (deg),dq0 components.Stator voltage  vd (pu),dq0 components.Stator voltage  vq (pu),Output reactive power  Qeo (pu)"
  "Delta Pa PSS 16 " : spsGenericPowerSystemStabilizerLib/Generic Power System Stabilizer  Tsensor=15e-3  K=2.5*1.25  Twashout=1  Tleadlag1=[60e-3 1]  Tleadlag2=[0 0]  VSlimits=[-0.15 0.15]  Vinit=0  Plot_On=off  MagdB_On=on  FreqRange=logspace(-2,2,500)
      settings: LibrarySourceBlock=|
      | sps_lib/Electrical Machines/Synchronous Machine Control/Generic
      | Power System Stabilizer
  Delta w PSS (Kundur) 16 : spsGenericPowerSystemStabilizerLib/Generic Power System Stabilizer  Tsensor=15e-3  K=30  Twashout=10  Tleadlag1=[50e-3 20e-3]  Tleadlag2=[3 5.4]  VSlimits=[-0.15 0.15]  Vinit=0  Plot_On=off  MagdB_On=on  FreqRange=logspace(-2,2,500)
      settings: LibrarySourceBlock=|
      | sps_lib/Electrical Machines/Synchronous Machine Control/Generic
      | Power System Stabilizer
  EXCITATION16 : spsExcitationSystemLib/Excitation System  tr=AVR_Data(13,1)  reg=[ AVR_Data(13,2:3) ]  exc=[ 1, 0 ]  tgr=[ AVR_Data(13,4:5)]  damp=[ 0, 0 ]  sat=[ 0, 0 ]  lim="[ AVR_Data(13,7:8)  0 ]"  v0=[1 1.0014]
      settings: LibrarySourceBlock=sps_lib/Electrical Machines/Synchronous Machine Control/Excitation System
  MB-PSS16 : spsMultiBandPowerSystemStabilizerLib/Multi-Band Power System Stabilizer  OperationMode=Simplified settings  Kg=MB(1)  GL=[MB(2) MB(3)]  GI=[MB(4) MB(5)]  GH=[MB(6) MB(7)]  GLd=[66 66 9.4]  TcLF=[1.667 2 0 0 0 0 2 2.4 0 0 0 0 1 1]  GId=[66 66 47.6]  TcIF=[1 1 0.25 0.3 0 0 1 1 0.3 0.36 0 0 0 0]  GHd=[66 66 233]  TcHF="[0.01 0.012 0 0 0 0  0.012 0.0144 0 0 0 0 1 1]"  LIM=[.075 .15 .15 .15]  Plot_On=off  MagdB_On=off  FreqRange=logspace(-2,2,500)
      settings: LibrarySourceBlock=|
      | sps_lib/Electrical Machines/Synchronous Machine Control/Multi-Band
      | Power System Stabilizer
  Multiport Switch1 : MultiPortSwitch  Inputs=4  SaturateOnIntegerOverflow=off
  PSS model3 : Constant  Value=0
  PSS model4 : Constant
  Real-Imag to Complex1 : RealImagToComplex
  STG13 : spsSteamTurbineandGovernorLib/Steam Turbine and Governor  gentype=Tandem-compound (single mass)  reg1="[ 1  0.05    0 ]"  reg2="[ 0.001  0.15 ]"  reg3="[ -0.1  0.1  0  4.496 ]"  N=Ns  turb1="[ 0  10   3.3   0.5   ]"  turb2="[   0   0.36    0.36   0.28   ]"  HA="[ 0.046  1.430  1.465   0.192 ]"  KA="[ 90.44  53.88  64.59   62.94  ]"  DA="[ 0.0115  0.3575  0.3663   0.0137  ]"  ini1=0.58333  ini2=[0.779316,-31.4247]
      settings: LibrarySourceBlock=|
      | sps_lib/Electrical Machines/Synchronous Machine Control/Steam Turbine
      | and Governor
  Sum2 : Sum  InputSameDT=on  SaturateOnIntegerOverflow=on  OutDataTypeStr=Inherit: Same as first input
  Sum3 : Sum  Inputs=-+  InputSameDT=on  SaturateOnIntegerOverflow=on  OutDataTypeStr=Inherit: Same as first input
  Terminator3 : Terminator
  Terminator4 : Terminator
  Terminator5 : Terminator
  wref16 : Constant
  Pm16 : Outport  InitialOutput=0
  Vf16 : Outport  Port=2  InitialOutput=0
  tag scope: EFD16=global, Pa16=global, Pe16=global, Q16=global, Vt16=global, d_theta16=global, pss16=global, theta16=global, w16=global
  wires:
  PSS16/1 -> Sum2/1
  Multiport Switch1/1 -> EXCITATION16/4, [pss16]
  PSS model3/1 -> Multiport Switch1/2
  MB-PSS16/1 -> Multiport Switch1/3
  Delta w PSS (Kundur) 16/1 -> Multiport Switch1/4
  "Delta Pa PSS 16 "/1 -> Multiport Switch1/5
  PSS model4/1 -> Sum2/2
  Sum2/1 -> Multiport Switch1/1
  Sum3/1 -> "Delta Pa PSS 16 "/1, [Pa16]  "Pm-Pe"
  Bus Selector/8 -> [Q16]  "<Output reactive power  Qeo (pu)>"
  Bus Selector/4 -> MB-PSS16/1, Delta w PSS (Kundur) 16/1  "<Rotor speed deviation  dw (pu)>"
  Bus Selector/3 -> [Pe16], Sum3/1  "<Electrical power  Pe (pu)>"
  Bus Selector/2 -> [d_theta16], STG13/4  "<Rotor angle deviation  d_theta (rad)>"
  Bus Selector/1 -> STG13/3, [w16]  "<Rotor speed  wm  (pu)>"
  STG13/1 -> Terminator5/1
  STG13/2 -> Terminator4/1
  STG13/4 -> Pm16/1, Sum3/2
  STG13/3 -> Terminator3/1
  Bus Selector/6 -> Real-Imag to Complex1/1, EXCITATION16/2  "<Stator voltage  vd (pu)>"
  Bus Selector/5 -> [theta16]  "<Rotor mechanical angle  theta (deg)>"
  Real-Imag to Complex1/1 -> [Vt16]
  EXCITATION16/1 -> [EFD16], Vf16/1
  Vref16/1 -> EXCITATION16/1
  m16/1 -> Bus Selector/1
  Pref16/1 -> STG13/2
  wref16/1 -> STG13/1
  Bus Selector/7 -> Real-Imag to Complex1/2, EXCITATION16/3  "<Stator voltage  vq (pu)>"
